simulink model "PV_Wind_BESS_10kV_R2026a"  (R2026a)
settings: Solver=ode23t  StopTime=0.2  MaxStep=1e-4
InitFcn:
  | run(fullfile(fileparts(get_param(bdroot,'FileName')),'..','scripts','init_10kv_architecture.m'));
undefined symbols (not defined in the file): P
libraries: ee_lib x18, fl_lib x3, nesl_utility x1
settings Model: Creator=fakebob2004  LastModifiedBy=fakebob2004
settings SimscapeCC: SimscapeLogType=none

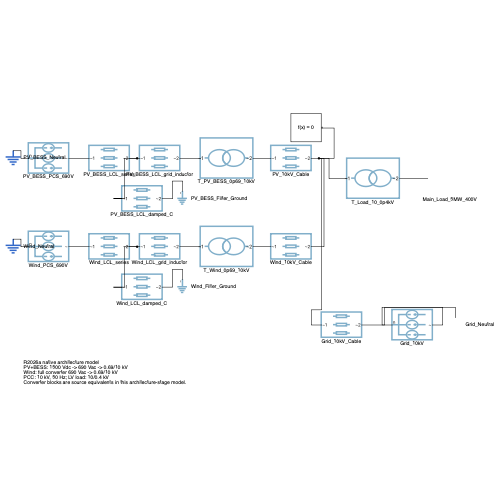
[thumbnail: Simulink's stored preview of the top-level diagram]
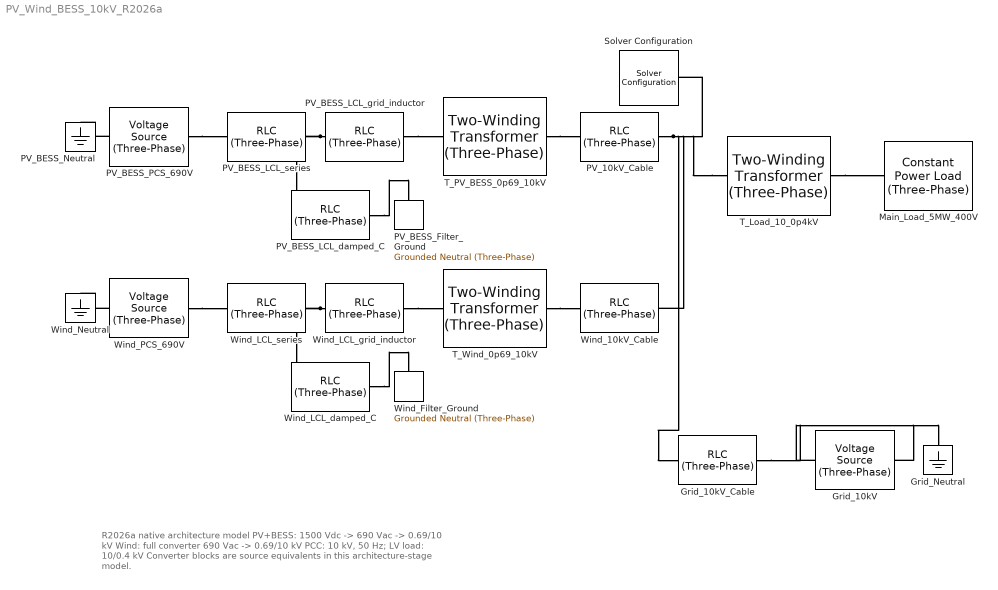
== system PV_Wind_BESS_10kV_R2026a ==
  note: R2026a native architecture model
      | PV+BESS: 1500 Vdc -> 690 Vac -> 0.69/10 kV
      | Wind: full converter 690 Vac -> 0.69/10 kV
      | PCC: 10 kV, 50 Hz; LV load: 10/0.4 kV
      | Converter blocks are source equivalents in this architecture-stage model.
  Grid_10kV : ee_lib/Sources/Voltage Source (Three-Phase)  vline_rms=P.grid.Vll_V V  shift=0 deg  freq=P.meta.frequency_Hz Hz  impedance_option=1  SShortCircuit=P.grid.short_circuit_VA A*V  XR=P.grid.XR  R=0.01 Ohm  L=3.97e-4 H  harmonic_option=0  harmonic_orders=[5, 7, 11, 13]  harmonic_ratios=[.1, .1, .1, .1]  G_parasitic=0 1/Ohm  I_specify=off  I_priority=None  I=[0, 0, 0] A  I_nominal_specify=off  I_nominal_value=1  I_nominal_unit=A
  Grid_10kV_Cable : ee_lib/Passive/RLC Assemblies/RLC (Three-Phase)  port_option=ee.enum.threePhasePort.composite  component_structure=ee.enum.rlc.structure.SeriesRL  R=P.line.grid.R_ohm Ohm  L=P.line.grid.L_H H  C=1e-6 F  R_parasitic=0 Ohm  G_parasitic=0 1/Ohm  IL_specify=off  IL_priority=High  IL=[0, 0, 0] A  IL_nominal_specify=off  IL_nominal_value=1  IL_nominal_unit=A  VC_specify=off  VC_priority=High  VC=[0, 0, 0] V  VC_nominal_specify=off  VC_nominal_value=1  VC_nominal_unit=V
  Grid_Neutral : fl_lib/Electrical/Electrical Elements/Electrical Reference
  Main_Load_5MW_400V : ee_lib/Passive/Constant Power Load (Three-Phase)  port_option=ee.enum.threePhasePort.composite  FRated=P.meta.frequency_Hz Hz  active_power=P.rating.main_load_W W  reactive_power=0 A*kV  Vline_rms_min=0.7*P.base.V400_V V  tau=0.01 s  Vline_rms_ini=P.base.V400_V V  Vang_ini=0 deg  gmin=1e-6 S
  PV_10kV_Cable : ee_lib/Passive/RLC Assemblies/RLC (Three-Phase)  port_option=ee.enum.threePhasePort.composite  component_structure=ee.enum.rlc.structure.SeriesRL  R=P.line.pv.R_ohm Ohm  L=P.line.pv.L_H H  C=1e-6 F  R_parasitic=0 Ohm  G_parasitic=0 1/Ohm  IL_specify=off  IL_priority=High  IL=[0, 0, 0] A  IL_nominal_specify=off  IL_nominal_value=1  IL_nominal_unit=A  VC_specify=off  VC_priority=High  VC=[0, 0, 0] V  VC_nominal_specify=off  VC_nominal_value=1  VC_nominal_unit=V
  PV_BESS_Filter_Ground : ee_lib/Connectors & References/Grounded Neutral (Three-Phase)  port_option=ee.enum.threePhasePort.composite
  PV_BESS_LCL_damped_C : ee_lib/Passive/RLC Assemblies/RLC (Three-Phase)  port_option=ee.enum.threePhasePort.composite  component_structure=ee.enum.rlc.structure.SeriesRC  R=P.filter.Rd_ohm Ohm  L=1e-3 H  C=P.filter.C_F F  R_parasitic=0 Ohm  G_parasitic=0 1/Ohm  IL_specify=off  IL_priority=High  IL=[0, 0, 0] A  IL_nominal_specify=off  IL_nominal_value=1  IL_nominal_unit=A  VC_specify=off  VC_priority=High  VC=[0, 0, 0] V  VC_nominal_specify=off  VC_nominal_value=1  VC_nominal_unit=V
  PV_BESS_LCL_grid_inductor : ee_lib/Passive/RLC Assemblies/RLC (Three-Phase)  port_option=ee.enum.threePhasePort.composite  component_structure=ee.enum.rlc.structure.SeriesRL  R=P.filter.R2_ohm Ohm  L=P.filter.L2_H H  C=1e-6 F  R_parasitic=0 Ohm  G_parasitic=0 1/Ohm  IL_specify=off  IL_priority=High  IL=[0, 0, 0] A  IL_nominal_specify=off  IL_nominal_value=1  IL_nominal_unit=A  VC_specify=off  VC_priority=High  VC=[0, 0, 0] V  VC_nominal_specify=off  VC_nominal_value=1  VC_nominal_unit=V
  PV_BESS_LCL_series : ee_lib/Passive/RLC Assemblies/RLC (Three-Phase)  port_option=ee.enum.threePhasePort.composite  component_structure=ee.enum.rlc.structure.SeriesRL  R=P.filter.R1_ohm Ohm  L=P.filter.L1_H H  C=1e-6 F  R_parasitic=0 Ohm  G_parasitic=0 1/Ohm  IL_specify=off  IL_priority=High  IL=[0, 0, 0] A  IL_nominal_specify=off  IL_nominal_value=1  IL_nominal_unit=A  VC_specify=off  VC_priority=High  VC=[0, 0, 0] V  VC_nominal_specify=off  VC_nominal_value=1  VC_nominal_unit=V
  PV_BESS_Neutral : fl_lib/Electrical/Electrical Elements/Electrical Reference
  PV_BESS_PCS_690V : ee_lib/Sources/Voltage Source (Three-Phase)  vline_rms=P.base.V690_V V  shift=30 deg  freq=P.meta.frequency_Hz Hz  impedance_option=1  SShortCircuit=20*P.rating.unit_converter_VA A*V  XR=10  R=0.01 Ohm  L=3.97e-4 H  harmonic_option=0  harmonic_orders=[5, 7, 11, 13]  harmonic_ratios=[.1, .1, .1, .1]  G_parasitic=0 1/Ohm  I_specify=off  I_priority=None  I=[0, 0, 0] A  I_nominal_specify=off  I_nominal_value=1  I_nominal_unit=A
  Solver Configuration : nesl_utility/Solver Configuration  PhysicalDomain=network_engine_domain  SubClassName=solver  LeftPortType=input  RightPortType=generic  Tones=[]  Harmonics=[]  SimulateNoise=off  Profile=off  UseLocalSampling=off  EnableSwitchedLinearOptims=on  FrequencyDomain=off  UseCCode=off  RelTol=0.001  AbsTol=0.001  MinStep=1e-09  ToWorkspace=off  RevertToSquareIcSolve=off  NumHomotopyIterations=100  PhasorMode=off  PhasorModeNumHarmonics=1  ConsistencySolver=NEWTON_XTOL_AFTER_FTOL  CanonicalOrdering=CANONICAL  OptimizeIntermediates=OPTIMIZED  IndexReductionMethod=DerivativeReplacement  DoDC=off  ResidualTolerance=1e-09  ConsistencyTolSource=GLOBAL  ConsistencyAbsTol=0.001  ConsistencyRelTol=0.001  ConsistencyTolFactor=0.001  UseLocalSolver=off  LocalSolverChoice=NE_BACKWARD_EULER_ADVANCER  ResolveIndetEquations=on  FunctionEvalNumThread=1  LocalSolverSampleTime=0.001  DoFixedCost=off  MaxNonlinIter=3  MaxModeIter=2  ComputeImpulses=off  ImpulseIterations=2  LinearAlgebra=auto  LinearAlgebraNumThread=0  EquationFormulation=NE_TIME_EF  DelaysMemoryBudget=1024  AutomaticFiltering=on  FilteringTimeConstant=0.001  PartitionStorageMethod=AS_NEEDED  PartitionMemoryBudget=1024  PartitionMethod=ROBUST  MultibodyUseLocalSolver=off  MultibodyLocalSolverChoice=ODE1  MultibodyLocalSolverSampleTime=0.001
  T_Load_10_0p4kV : ee_lib/Passive/Transformers/Two-Winding Transformer (Three-Phase)  SRated=P.transformer.load.S_VA A*V  FRated=P.meta.frequency_Hz Hz  Winding1Connection=ee.enum.windingconnection.delta1  VRated1=P.transformer.load.Vhigh_V V  Winding2Connection=ee.enum.windingconnection.Yg  VRated2=P.transformer.load.Vlow_V V  CoreType=ee.enum.coretype.threelimb  pu_Rw1=P.transformer.load.pu_Rw1  pu_Rw2=P.transformer.load.pu_Rw2  leakage_reactance_option=ee.enum.transformer_leakage.include  pu_Xl1=P.transformer.load.pu_Xl1  pu_Xl2=P.transformer.load.pu_Xl2  magnetizing_resistance_option=ee.enum.transformer_magnetizingResistance.exclude  pu_Rm=500  magnetizing_reactance_option=ee.enum.transformer_magnetizingReactance.exclude  saturation_option=ee.enum.transformer_saturation.exclude  pu_Xm=500  current_data=[0, .002, 1, 2]  magnetic_flux_data=[0, 1.2, 1.5, 1.51]  pu_X0=0.5  i1_specify=off  i1_priority=None  i1=[0, 0, 0] A  i1_nominal_specify=off  i1_nominal_value=1  i1_nominal_unit=A  i2_specify=off  i2_priority=None  i2=[0, 0, 0] A  i2_nominal_specify=off  i2_nominal_value=1  i2_nominal_unit=A  phi_specify=off  phi_priority=None  phi=[0, 0, 0]  phi_nominal_specify=off  phi_nominal_value=1  phi_nominal_unit=1
  T_PV_BESS_0p69_10kV : ee_lib/Passive/Transformers/Two-Winding Transformer (Three-Phase)  SRated=P.transformer.unit.S_VA A*V  FRated=P.meta.frequency_Hz Hz  Winding1Connection=ee.enum.windingconnection.delta1  VRated1=P.transformer.unit.Vlow_V V  Winding2Connection=ee.enum.windingconnection.Yg  VRated2=P.transformer.unit.Vhigh_V V  CoreType=ee.enum.coretype.threelimb  pu_Rw1=P.transformer.unit.pu_Rw1  pu_Rw2=P.transformer.unit.pu_Rw2  leakage_reactance_option=ee.enum.transformer_leakage.include  pu_Xl1=P.transformer.unit.pu_Xl1  pu_Xl2=P.transformer.unit.pu_Xl2  magnetizing_resistance_option=ee.enum.transformer_magnetizingResistance.exclude  pu_Rm=500  magnetizing_reactance_option=ee.enum.transformer_magnetizingReactance.exclude  saturation_option=ee.enum.transformer_saturation.exclude  pu_Xm=500  current_data=[0, .002, 1, 2]  magnetic_flux_data=[0, 1.2, 1.5, 1.51]  pu_X0=0.5  i1_specify=off  i1_priority=None  i1=[0, 0, 0] A  i1_nominal_specify=off  i1_nominal_value=1  i1_nominal_unit=A  i2_specify=off  i2_priority=None  i2=[0, 0, 0] A  i2_nominal_specify=off  i2_nominal_value=1  i2_nominal_unit=A  phi_specify=off  phi_priority=None  phi=[0, 0, 0]  phi_nominal_specify=off  phi_nominal_value=1  phi_nominal_unit=1
  T_Wind_0p69_10kV : ee_lib/Passive/Transformers/Two-Winding Transformer (Three-Phase)  SRated=P.transformer.unit.S_VA A*V  FRated=P.meta.frequency_Hz Hz  Winding1Connection=ee.enum.windingconnection.delta1  VRated1=P.transformer.unit.Vlow_V V  Winding2Connection=ee.enum.windingconnection.Yg  VRated2=P.transformer.unit.Vhigh_V V  CoreType=ee.enum.coretype.threelimb  pu_Rw1=P.transformer.unit.pu_Rw1  pu_Rw2=P.transformer.unit.pu_Rw2  leakage_reactance_option=ee.enum.transformer_leakage.include  pu_Xl1=P.transformer.unit.pu_Xl1  pu_Xl2=P.transformer.unit.pu_Xl2  magnetizing_resistance_option=ee.enum.transformer_magnetizingResistance.exclude  pu_Rm=500  magnetizing_reactance_option=ee.enum.transformer_magnetizingReactance.exclude  saturation_option=ee.enum.transformer_saturation.exclude  pu_Xm=500  current_data=[0, .002, 1, 2]  magnetic_flux_data=[0, 1.2, 1.5, 1.51]  pu_X0=0.5  i1_specify=off  i1_priority=None  i1=[0, 0, 0] A  i1_nominal_specify=off  i1_nominal_value=1  i1_nominal_unit=A  i2_specify=off  i2_priority=None  i2=[0, 0, 0] A  i2_nominal_specify=off  i2_nominal_value=1  i2_nominal_unit=A  phi_specify=off  phi_priority=None  phi=[0, 0, 0]  phi_nominal_specify=off  phi_nominal_value=1  phi_nominal_unit=1
  Wind_10kV_Cable : ee_lib/Passive/RLC Assemblies/RLC (Three-Phase)  port_option=ee.enum.threePhasePort.composite  component_structure=ee.enum.rlc.structure.SeriesRL  R=P.line.wind.R_ohm Ohm  L=P.line.wind.L_H H  C=1e-6 F  R_parasitic=0 Ohm  G_parasitic=0 1/Ohm  IL_specify=off  IL_priority=High  IL=[0, 0, 0] A  IL_nominal_specify=off  IL_nominal_value=1  IL_nominal_unit=A  VC_specify=off  VC_priority=High  VC=[0, 0, 0] V  VC_nominal_specify=off  VC_nominal_value=1  VC_nominal_unit=V
  Wind_Filter_Ground : ee_lib/Connectors & References/Grounded Neutral (Three-Phase)  port_option=ee.enum.threePhasePort.composite
  Wind_LCL_damped_C : ee_lib/Passive/RLC Assemblies/RLC (Three-Phase)  port_option=ee.enum.threePhasePort.composite  component_structure=ee.enum.rlc.structure.SeriesRC  R=P.filter.Rd_ohm Ohm  L=1e-3 H  C=P.filter.C_F F  R_parasitic=0 Ohm  G_parasitic=0 1/Ohm  IL_specify=off  IL_priority=High  IL=[0, 0, 0] A  IL_nominal_specify=off  IL_nominal_value=1  IL_nominal_unit=A  VC_specify=off  VC_priority=High  VC=[0, 0, 0] V  VC_nominal_specify=off  VC_nominal_value=1  VC_nominal_unit=V
  Wind_LCL_grid_inductor : ee_lib/Passive/RLC Assemblies/RLC (Three-Phase)  port_option=ee.enum.threePhasePort.composite  component_structure=ee.enum.rlc.structure.SeriesRL  R=P.filter.R2_ohm Ohm  L=P.filter.L2_H H  C=1e-6 F  R_parasitic=0 Ohm  G_parasitic=0 1/Ohm  IL_specify=off  IL_priority=High  IL=[0, 0, 0] A  IL_nominal_specify=off  IL_nominal_value=1  IL_nominal_unit=A  VC_specify=off  VC_priority=High  VC=[0, 0, 0] V  VC_nominal_specify=off  VC_nominal_value=1  VC_nominal_unit=V
  Wind_LCL_series : ee_lib/Passive/RLC Assemblies/RLC (Three-Phase)  port_option=ee.enum.threePhasePort.composite  component_structure=ee.enum.rlc.structure.SeriesRL  R=P.filter.R1_ohm Ohm  L=P.filter.L1_H H  C=1e-6 F  R_parasitic=0 Ohm  G_parasitic=0 1/Ohm  IL_specify=off  IL_priority=High  IL=[0, 0, 0] A  IL_nominal_specify=off  IL_nominal_value=1  IL_nominal_unit=A  VC_specify=off  VC_priority=High  VC=[0, 0, 0] V  VC_nominal_specify=off  VC_nominal_value=1  VC_nominal_unit=V
  Wind_Neutral : fl_lib/Electrical/Electrical Elements/Electrical Reference
  Wind_PCS_690V : ee_lib/Sources/Voltage Source (Three-Phase)  vline_rms=P.base.V690_V V  shift=30 deg  freq=P.meta.frequency_Hz Hz  impedance_option=1  SShortCircuit=20*P.rating.unit_converter_VA A*V  XR=10  R=0.01 Ohm  L=3.97e-4 H  harmonic_option=0  harmonic_orders=[5, 7, 11, 13]  harmonic_ratios=[.1, .1, .1, .1]  G_parasitic=0 1/Ohm  I_specify=off  I_priority=None  I=[0, 0, 0] A  I_nominal_specify=off  I_nominal_value=1  I_nominal_unit=A
  connections:
  PV_BESS_PCS_690V/LConn1 -- PV_BESS_Neutral/LConn1
  PV_BESS_PCS_690V/RConn1 -- PV_BESS_LCL_series/LConn1
  PV_BESS_LCL_grid_inductor/LConn1 -- PV_BESS_LCL_series/RConn1 -- PV_BESS_LCL_damped_C/LConn1
  PV_BESS_LCL_damped_C/RConn1 -- PV_BESS_Filter_Ground/LConn1
  PV_BESS_LCL_grid_inductor/RConn1 -- T_PV_BESS_0p69_10kV/LConn1
  T_PV_BESS_0p69_10kV/RConn1 -- PV_10kV_Cable/LConn1
  Wind_PCS_690V/LConn1 -- Wind_Neutral/LConn1
  Wind_PCS_690V/RConn1 -- Wind_LCL_series/LConn1
  Wind_LCL_grid_inductor/LConn1 -- Wind_LCL_series/RConn1 -- Wind_LCL_damped_C/LConn1
  Wind_LCL_damped_C/RConn1 -- Wind_Filter_Ground/LConn1
  Wind_LCL_grid_inductor/RConn1 -- T_Wind_0p69_10kV/LConn1
  T_Wind_0p69_10kV/RConn1 -- Wind_10kV_Cable/LConn1
  Grid_10kV_Cable/RConn1 -- Grid_10kV/RConn1
  Grid_10kV/LConn1 -- Grid_Neutral/LConn1
  T_Load_10_0p4kV/RConn1 -- Main_Load_5MW_400V/LConn1
  T_Load_10_0p4kV/LConn1 -- PV_10kV_Cable/RConn1 -- Wind_10kV_Cable/RConn1 -- Grid_10kV_Cable/LConn1 -- Solver Configuration/RConn1
